simulink model "Admittance_6D"  (R2025b)
settings: Solver=FixedStepDiscrete  StartTime=0.0  StopTime=4  FixedStep=0.002  RelTol=1e-3
settings Model: Creator=Compu  LastModifiedBy=Compu

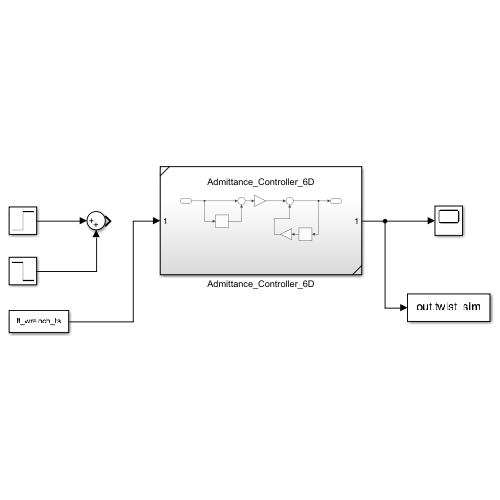
[thumbnail: Simulink's stored preview of the top-level diagram]
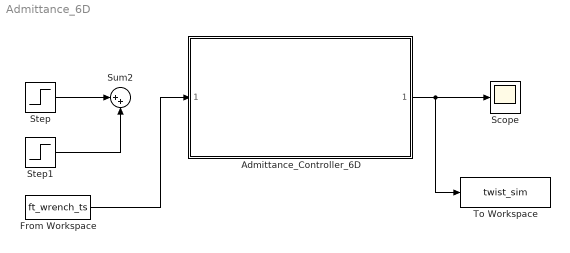
== system Admittance_6D ==
  Admittance_Controller_6D : Subsystem  ReferencedSubsystem=Admittance_Controller_6D
  From Workspace : FromWorkspace  VariableName=ft_wrench_ts
  Scope : Scope
      settings: ActiveDisplayYMinimum=-0.03027721724283244  ActiveDisplayYMaximum=0.04168394283405296
  Step : Step  Time=0.5  Before=zeros(6,1)  After=[5;0;0;0;0;0]  SampleTime=0.002
  Step1 : Step  Time=1.5  Before=zeros(6,1)  After=[-5;0;0;0;0;0]  SampleTime=0.002
  Sum2 : Sum  Inputs=|++
  To Workspace : ToWorkspace  VariableName=twist_sim  SaveFormat=Timeseries  SampleTime=-1
  wires:
  Step/1 -> Sum2/1
  Step1/1 -> Sum2/2
  Admittance_Controller_6D/1 -> Scope/1, To Workspace/1
  From Workspace/1 -> Admittance_Controller_6D/1
